simulink model "PE_Rectifier"  (R2025a)
settings: Solver=VariableStepAuto  StartTime=0.0  StopTime=1  FixedStep=1e-6  MaxStep=1e-6  RelTol=1e-4
libraries: spsDiodeLib x4, spsVoltageMeasurementLib x2, spsACVoltageSourceLib x1, spsSeriesRLCBranchLib x1, spspowerguiLib x1
settings Model: Creator=abhis  LastModifiedBy=abhis

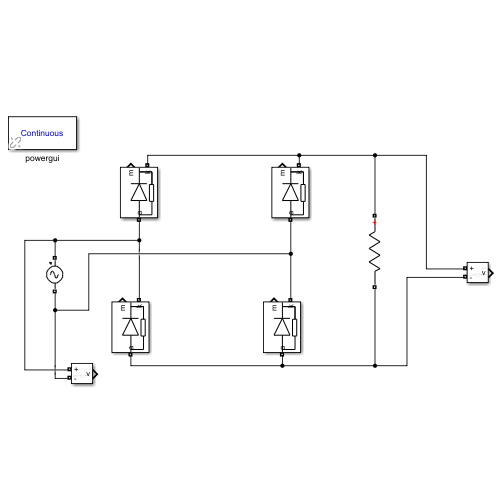
[thumbnail: Simulink's stored preview of the top-level diagram]
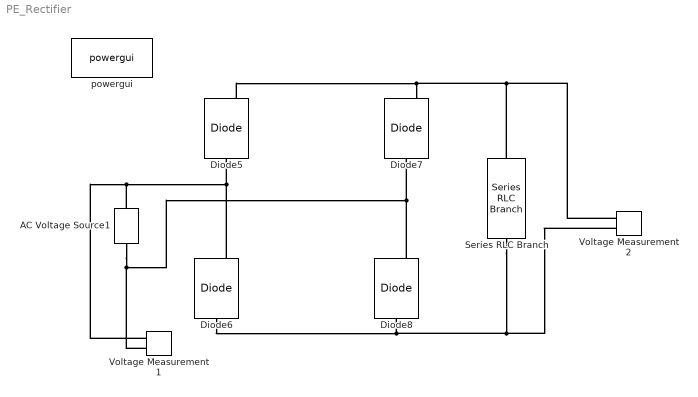
== system PE_Rectifier ==
  AC Voltage Source1 : spsACVoltageSourceLib/AC Voltage Source  Amplitude=30*sqrt(2)  Phase=0  Frequency=50  SampleTime=0  Measurements=None  BusType=swing  Pref=10e3  Qref=0  Qmin=-inf  Qmax=+inf
  Diode{5..8} (4 alike) : spsDiodeLib/Diode  Ron=0.001  Lon=0  Vf=0.8  IC=0  UseSnubber=0  Rs=500  Cs=250e-9  Measurements=on
  Series RLC Branch : spsSeriesRLCBranchLib/Series RLC Branch  LConnTagsString=__new0  RConnTagsString=__new0  BranchType=R  Resistance=1  Inductance=1e-3  SetiL0=off  InitialCurrent=0  Capacitance=1e-6  Setx0=off  InitialVoltage=0  Measurements=None
  Voltage Measurement1 : spsVoltageMeasurementLib/Voltage Measurement  PhasorSimulation=off  OutputType=Complex  PSBequivalent=0
  Voltage Measurement2 : spsVoltageMeasurementLib/Voltage Measurement  PhasorSimulation=off  OutputType=Complex  PSBequivalent=0
  powergui : spspowerguiLib/powergui  Priority=1  SimulationMode=Continuous  SampleTime=1e-6  frequency=50  Iterations=50  frequencyindice=50  Pbase=100e6  ErrMax=1e-4  UnitsV=kV  UnitsW=MW  buscounter=0  FunctionMessages=off  echomessages=off  EnableUseOfTLC=off  CurrentSourceSwitches=off  DisableSnubberDevices=off  DisableRonSwitches=off  DisableVfSwitches=off  DisplayEquations=off  AutomaticDiscreteSolvers=off  SolverType=Tustin/Backward Euler (TBE)  Interpol=off  ExternalGateDelay=off  methode=off  Ts=100  x0status=blocks  SPID=on  SwTol=0  HookPort=off  NonlinearTolerance=1e-4  nMaxIteration=100  ContinueOnMaxIteration=off  RestoreLinks=warning  ResistiveCurrentMeasurement=off  Frange=[0:2:500]  Ylog=off  Xlog=on  ShowGrid=off  save=off  variable=ZData  structure=0  ZoomFFT=off  StartTime=0.0  cycles=1  DisplayStyle=1  fundamental=60  FreqAxis=off  MaxFrequency=1000  frequencyindicesteady=1  RmsSteady=1  display=off
  connections:
  Diode7/RConn1 -- Series RLC Branch/LConn1 -- Voltage Measurement2/LConn1 -- Diode5/RConn1
  Diode7/LConn1 -- AC Voltage Source1/LConn1 -- Voltage Measurement1/LConn2 -- Diode8/RConn1
  Diode8/LConn1 -- Series RLC Branch/RConn1 -- Voltage Measurement2/LConn2 -- Diode6/LConn1
  Diode5/LConn1 -- Voltage Measurement1/LConn1 -- AC Voltage Source1/RConn1 -- Diode6/RConn1
